simulink model "ZoomActuatorControl_before_layout"  (R2026b)
settings: Solver=ode4  StopTime=12  FixedStep=0.01
model workspace (MAT data in the model file):
  disturbance1 = timeseries
  disturbance1.Name = 'unnamed'
  disturbance1.DataInfo = tsdata.datametadata
  disturbance1.DataInfo.Interpolation = tsdata.interpolation
  disturbance1.DataInfo.Interpolation.Fhandle : function handle (value not decoded)
  disturbance1.DataInfo.Interpolation.Name = 'linear'
  disturbance1.TimeInfo = tsdata.timemetadata
  disturbance1.TimeInfo.Length = 6
  disturbance1.TimeInfo.DuplicateTimes = 0
  disturbance1.TimeInfo.Time_ = [0; 6.99; 7; 7.49; 7.5; 12]
  disturbance1.TimeInfo.Initialized = 1
  disturbance1.QualityInfo = tsdata.qualmetadata
  disturbance1.Data_ = [0; 0; 0.03; 0.03; 0; 0]
  disturbance2 = timeseries
  disturbance2.Name = 'unnamed'
  disturbance2.DataInfo = tsdata.datametadata
  disturbance2.DataInfo.Interpolation = tsdata.interpolation
  disturbance2.DataInfo.Interpolation.Fhandle : function handle (value not decoded)
  disturbance2.DataInfo.Interpolation.Name = 'linear'
  disturbance2.TimeInfo = tsdata.timemetadata
  disturbance2.TimeInfo.Length = 6
  disturbance2.TimeInfo.DuplicateTimes = 0
  disturbance2.TimeInfo.Time_ = [0; 6.99; 7; 7.49; 7.5; 12]
  disturbance2.TimeInfo.Initialized = 1
  disturbance2.QualityInfo = tsdata.qualmetadata
  disturbance2.Data_ = [0; 0; -0.03; -0.03; 0; 0]
  focalBreakpoints = [70 75 80 85 90 95 100 105 110 115 120 125 130 135 140 145 150 155 160 165 170 175 180 185 190 195 200 205 210]
  focalCommand = timeseries
  focalCommand.Name = 'unnamed'
  focalCommand.DataInfo = tsdata.datametadata
  focalCommand.DataInfo.Interpolation = tsdata.interpolation
  focalCommand.DataInfo.Interpolation.Fhandle : function handle (value not decoded)
  focalCommand.DataInfo.Interpolation.Name = 'linear'
  focalCommand.TimeInfo = tsdata.timemetadata
  focalCommand.TimeInfo.Length = 4
  focalCommand.TimeInfo.DuplicateTimes = 0
  focalCommand.TimeInfo.Time_ = [0; 1.99; 2; 12]
  focalCommand.TimeInfo.Initialized = 1
  focalCommand.QualityInfo = tsdata.qualmetadata
  focalCommand.Data_ = [70; 70; 210; 210]
  gap1Table = [2.02367848331 2.87943028231 1.41582654433 6.74409771067 8.90084522258 8.94470794881 9.48943448775 10.1012670037 10.7186322219 11.312129679 11.8821048738 12.4231172215 12.9360755684 13.4224565664 13.883906037 14.321990023 14.7378563236 15.1338511735 15.5111104184 15.8709865113 16.215613706 16.5433796899 16.8581421692 17.1610547803 17.4494491161 17.728185185 17.996446295 18.2538789129 17.8693156943]
  group2Table = [43.537846057 41.6263743062 36.788319007 41.5287575368 41.9296794596 39.5861712588 38.0847711667 36.7942229245 35.6138964917 34.4935301619 33.4230326041 32.3883669373 31.3839952577 30.4061268335 29.4520205012 28.5192208644 27.6058185327 26.7110018773 25.8333152837 24.9717773211 24.1260566591 23.293581296 22.4754149381 21.6710859816 20.8776323867 20.0968053569 19.3272405678 18.5687173242 17.9193297313]
  initial1 = 2.02367848331
  initial2 = 43.537846057
libraries: sl_discontinuities x2
settings Model: Creator=hkawai  LastModifiedBy=hkawai

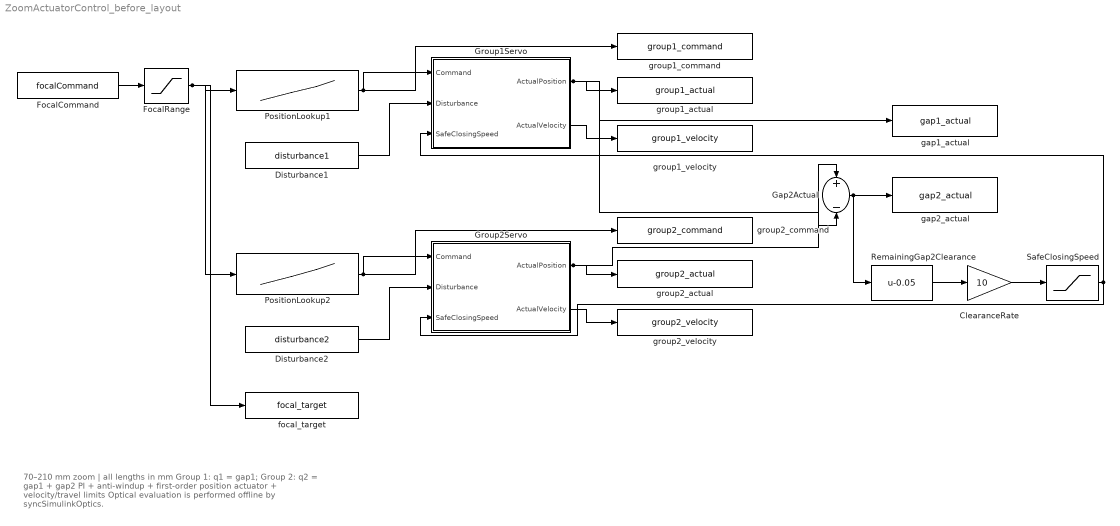
== system ZoomActuatorControl_before_layout ==
  note: 70–210 mm zoom | all lengths in mm
      | Group 1: q1 = gap1; Group 2: q2 = gap1 + gap2
      | PI + anti-windup + first-order position actuator + velocity/travel limits
      | Optical evaluation is performed offline by syncSimulinkOptics.
  ClearanceRate : Gain  Gain=10
  Disturbance1 : FromWorkspace  VariableName=disturbance1  Interpolate=off  OutputAfterFinalValue=Holding final value
  Disturbance2 : FromWorkspace  VariableName=disturbance2  Interpolate=off  OutputAfterFinalValue=Holding final value
  FocalCommand : FromWorkspace  VariableName=focalCommand  Interpolate=off  OutputAfterFinalValue=Holding final value
  FocalRange : Saturate  UpperLimit=210  LowerLimit=70
  Gap2Actual : Sum  Inputs=+-
  Group1Servo : Subsystem
  Group2Servo : Subsystem
  PositionLookup1 : Lookup_n-D  NumberOfTableDimensions=1  BreakpointsForDimension1=focalBreakpoints  Table=gap1Table  InternalRulePriority=Speed  RndMeth=Simplest
  PositionLookup2 : Lookup_n-D  NumberOfTableDimensions=1  BreakpointsForDimension1=focalBreakpoints  Table=group2Table  InternalRulePriority=Speed  RndMeth=Simplest
  RemainingGap2Clearance : Bias  Bias=-0.05  SaturateOnIntegerOverflow=off
  SafeClosingSpeed : Saturate  UpperLimit=20  LowerLimit=0
  focal_target : ToWorkspace  VariableName=focal_target  SaveFormat=Timeseries  SampleTime=-1
  gap1_actual : ToWorkspace  VariableName=gap1_actual  SaveFormat=Timeseries  SampleTime=-1
  gap2_actual : ToWorkspace  VariableName=gap2_actual  SaveFormat=Timeseries  SampleTime=-1
  group1_actual : ToWorkspace  VariableName=group1_actual  SaveFormat=Timeseries  SampleTime=-1
  group1_command : ToWorkspace  VariableName=group1_command  SaveFormat=Timeseries  SampleTime=-1
  group1_velocity : ToWorkspace  VariableName=group1_velocity  SaveFormat=Timeseries  SampleTime=-1
  group2_actual : ToWorkspace  VariableName=group2_actual  SaveFormat=Timeseries  SampleTime=-1
  group2_command : ToWorkspace  VariableName=group2_command  SaveFormat=Timeseries  SampleTime=-1
  group2_velocity : ToWorkspace  VariableName=group2_velocity  SaveFormat=Timeseries  SampleTime=-1
  wires:
  FocalCommand/1 -> FocalRange/1
  FocalRange/1 -> PositionLookup1/1, PositionLookup2/1, focal_target/1
  PositionLookup1/1 -> Group1Servo/1(Command), group1_command/1
  Disturbance1/1 -> Group1Servo/2(Disturbance)
  Group1Servo/1(ActualPosition) -> group1_actual/1, Gap2Actual/2, gap1_actual/1
  Group1Servo/2(ActualVelocity) -> group1_velocity/1
  PositionLookup2/1 -> Group2Servo/1(Command), group2_command/1
  Disturbance2/1 -> Group2Servo/2(Disturbance)
  Group2Servo/1(ActualPosition) -> group2_actual/1, Gap2Actual/1
  Group2Servo/2(ActualVelocity) -> group2_velocity/1
  Gap2Actual/1 -> RemainingGap2Clearance/1, gap2_actual/1
  RemainingGap2Clearance/1 -> ClearanceRate/1
  ClearanceRate/1 -> SafeClosingSpeed/1
  SafeClosingSpeed/1 -> Group1Servo/3(SafeClosingSpeed), Group2Servo/3(SafeClosingSpeed)

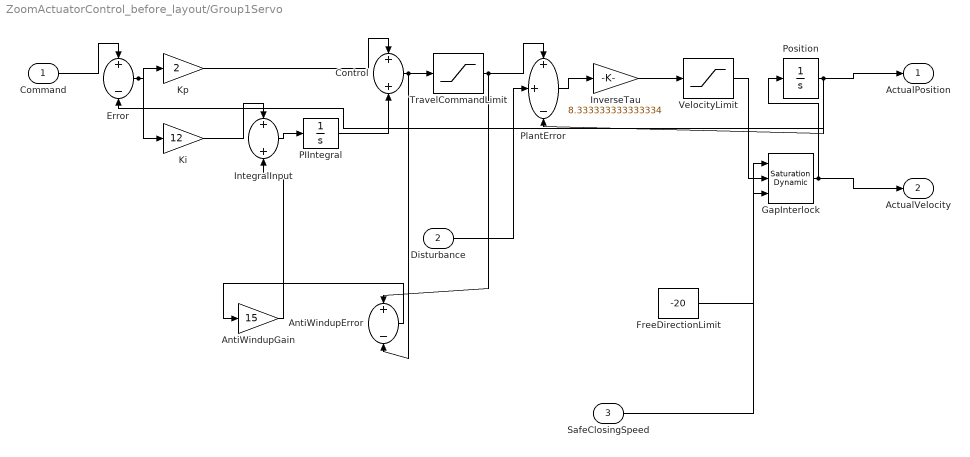
== system ZoomActuatorControl_before_layout/Group1Servo ==
  Command : Inport
  Disturbance : Inport  Port=2
  SafeClosingSpeed : Inport  Port=3
  AntiWindupError : Sum  Inputs=+-
  AntiWindupGain : Gain  Gain=15
  Control : Sum
  Error : Sum  Inputs=+-
  FreeDirectionLimit : Constant  Value=-20
  GapInterlock : sl_discontinuities/Saturation Dynamic  OutMin=[]  OutMax=[]  OutDataTypeStr=Inherit: Same as second input  OutDataType=fixdt(1, 16)  OutScaling=2^-10  DoSatur=off
      settings: LibrarySourceBlock=|
      | simulink/Discontinuities/Saturation
      | Dynamic
  IntegralInput : Sum
  InverseTau : Gain  Gain=8.333333333333334
  Ki : Gain  Gain=12
  Kp : Gain  Gain=2
  PIIntegral : Integrator  InitialCondition=initial1
  PlantError : Sum  Inputs=++-
  Position : Integrator  InitialCondition=initial1  LimitOutput=on  UpperSaturationLimit=18.25387891290362  LowerSaturationLimit=1.41582654432993
  TravelCommandLimit : Saturate  UpperLimit=18.25387891290362  LowerLimit=1.41582654432993
  VelocityLimit : Saturate  UpperLimit=20  LowerLimit=-20
  ActualPosition : Outport
  ActualVelocity : Outport  Port=2
  wires:
  SafeClosingSpeed/1 -> GapInterlock/1
  FreeDirectionLimit/1 -> GapInterlock/3
  Command/1 -> Error/1
  Position/1 -> Error/2, PlantError/3, ActualPosition/1
  Error/1 -> Kp/1, Ki/1
  Ki/1 -> IntegralInput/1
  IntegralInput/1 -> PIIntegral/1
  Kp/1 -> Control/1
  PIIntegral/1 -> Control/2
  Control/1 -> TravelCommandLimit/1, AntiWindupError/2
  TravelCommandLimit/1 -> AntiWindupError/1, PlantError/1
  AntiWindupError/1 -> AntiWindupGain/1
  AntiWindupGain/1 -> IntegralInput/2
  Disturbance/1 -> PlantError/2
  PlantError/1 -> InverseTau/1
  InverseTau/1 -> VelocityLimit/1
  VelocityLimit/1 -> GapInterlock/2
  GapInterlock/1 -> Position/1, ActualVelocity/1

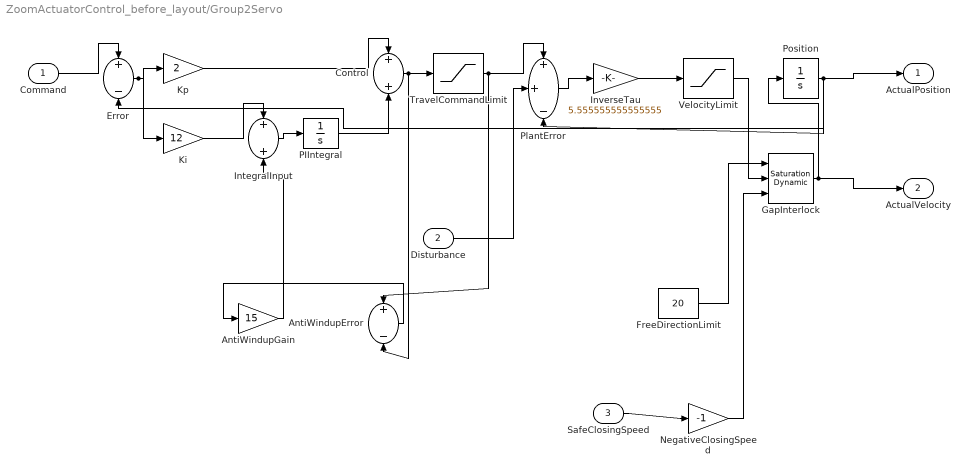
== system ZoomActuatorControl_before_layout/Group2Servo ==
  Command : Inport
  Disturbance : Inport  Port=2
  SafeClosingSpeed : Inport  Port=3
  AntiWindupError : Sum  Inputs=+-
  AntiWindupGain : Gain  Gain=15
  Control : Sum
  Error : Sum  Inputs=+-
  FreeDirectionLimit : Constant  Value=20
  GapInterlock : sl_discontinuities/Saturation Dynamic  OutMin=[]  OutMax=[]  OutDataTypeStr=Inherit: Same as second input  OutDataType=fixdt(1, 16)  OutScaling=2^-10  DoSatur=off
      settings: LibrarySourceBlock=|
      | simulink/Discontinuities/Saturation
      | Dynamic
  IntegralInput : Sum
  InverseTau : Gain  Gain=5.555555555555555
  Ki : Gain  Gain=12
  Kp : Gain  Gain=2
  NegativeClosingSpeed : Gain  Gain=-1
  PIIntegral : Integrator  InitialCondition=initial2
  PlantError : Sum  Inputs=++-
  Position : Integrator  InitialCondition=initial2  LimitOutput=on  UpperSaturationLimit=81.63080000000004  LowerSaturationLimit=17.91932973126335
  TravelCommandLimit : Saturate  UpperLimit=81.63080000000004  LowerLimit=17.91932973126335
  VelocityLimit : Saturate  UpperLimit=20  LowerLimit=-20
  ActualPosition : Outport
  ActualVelocity : Outport  Port=2
  wires:
  SafeClosingSpeed/1 -> NegativeClosingSpeed/1
  FreeDirectionLimit/1 -> GapInterlock/1
  NegativeClosingSpeed/1 -> GapInterlock/3
  Command/1 -> Error/1
  Position/1 -> Error/2, PlantError/3, ActualPosition/1
  Error/1 -> Kp/1, Ki/1
  Ki/1 -> IntegralInput/1
  IntegralInput/1 -> PIIntegral/1
  Kp/1 -> Control/1
  PIIntegral/1 -> Control/2
  Control/1 -> TravelCommandLimit/1, AntiWindupError/2
  TravelCommandLimit/1 -> AntiWindupError/1, PlantError/1
  AntiWindupError/1 -> AntiWindupGain/1
  AntiWindupGain/1 -> IntegralInput/2
  Disturbance/1 -> PlantError/2
  PlantError/1 -> InverseTau/1
  InverseTau/1 -> VelocityLimit/1
  VelocityLimit/1 -> GapInterlock/2
  GapInterlock/1 -> Position/1, ActualVelocity/1
